simulink model "afe_rst_inv_psm_distributed_control_two_delays"  (R2026a)
settings: Solver=ode1be  StopTime=simlength  FixedStep=tc  MaxStep=Tc
values from neighbouring files (symbols this model uses):
  Amplitude_U = 1.16    [grid_fault_generator.m]
  Amplitude_V = Amplitude_U    (= 1.16)    [grid_fault_generator.m]
  Amplitude_W = Amplitude_U    (= 1.16)    [grid_fault_generator.m]
  end_time_LVRT = start_time_LVRT + error_length    [grid_fault_generator.m]
  Igrid_phase_normalization_factor = 270*sqrt(2)    [grid_emulator.m]
  omega_grid_emulator_nom = w_grid    (= 314.159265359)    [grid_emulator.m]
  omega_grid_nom = w_grid    (= 314.159265359)    [grid_emulator.m]
  t_ramp = 20e-3    (= 0.02)    [grid_fault_generator.m]
  ugrid_factor = 1    [grid_emulator.m]
  V_phase_normalization_factor = Vgrid_phase_normalization_factor    [grid_emulator.m]
  Vdc_bez = 1070    [grid_emulator.m]
  Vemu_ref_norm = Vemu_ref * sqrt(2) / V_phase_normalization_factor    [grid_emulator.m]
  vn_eta_pu = 0    [grid_emulator.m]
  vn_xi_pu = 0    [grid_emulator.m]
  vp_xi_pu = 1    [grid_emulator.m]
undefined symbols (not defined in the file or in its folder): Adrso, Aresd, Bresd, CFi, CFu, Cresd, Crso, CTRPIFF_CLIP_RELEASE, dead_time_INV, emf_fb_p, emf_fb_p_ccaller_1, emf_fb_p_ccaller_2, emf_p, emf_p_ccaller_1, emf_p_ccaller_2, fPWM_INV, g0_161Hz, g0_500Hz, g1_161Hz, g1_500Hz, i_grid_neg_eta_lim, i_grid_neg_eta_red_lim, i_grid_neg_xi_lim, i_grid_neg_xi_red_lim, i_grid_pos_eta_lim, i_grid_pos_eta_red_lim, ibez, id_lim, ieta_neg_ref_lim, ieta_pos_ref_lim, iq_lim, ixi_pos_ref_lim, Jm_norm, k_frt_ref, kg, ki_afe, ki_i, ki_id, ki_iq, ki_rc_neg_grid, ki_rc_pos_grid, ki_vs, ki_w, kp_afe, kp_i, kp_id, kp_iq, kp_rc_neg_grid, kp_rc_pos_grid, kp_vs, kp_w, kw, l1, l2, Lalpha_norm, Ld_norm, Ldrso, Lq_norm, Ls_norm, luenberger_l1 ... (+30)
libraries: fl_lib x146, nesl_utility x62, simulink x8, cstblocks_lti x7, sl_discontinuities x3, single_phase_transformer_lib x3, flexshaft_lib x1, permanent_magnet_synchronous_machine x1
(part 1 of 14)
settings Model: SimulationMode=accelerator  Creator=dbagn  LastModifiedBy=dbagn
settings SolverCC: NumberNewtonIterations=3.0  ZeroCrossControl=DisableAll  SolverResetMethod=Robust
settings SFSimCC: SimUserIncludeDirs=include  CustomCodeUndefinedFunction=ThrowError
settings SFSimCC: SimCustomHeaderCode=|
  | #include "mavgflt.h"
  | #include "mavgflt_simulink.h"
  | #include "bemf_obsv_load_est.h"
  | #include "bemf_obsv.h"
  | #include "bemf_obsv_simulink.h"
  | #include "dqvector_pi.h"
  | #include "dqvector_pi_simulink.h"
  | #include "bemf_obsv_load_est_simulink.h"
  | #include "sv_pwm.h"
  | #include "sv_pwm_simulink.h"
settings SFSimCC: SimUserSources=|
  | "mavgflt_simulink.c"
  | "mavgflt.c"
  | "bemf_obsv_simulink.c"
  | "bemf_obsv.c"
  | "bemf_obsv_load_est_simulink.c"
  | "bemf_obsv_load_est.c"
  | "dqvector_pi.c"
  | "dqvector_pi_simulink.c"
  | "sv_pwm_simulink.c"
  | "sv_pwm.c"
settings SimscapeCC: SimscapeNominalValues="[{\"value\":\"1\",\"unit\":\"A\"},{\"value\":\"1\",\"unit\":\"bar\"},{\"value\":\"1\",\"unit\":\"cm^2\"},{\"value\":\"1\",\"unit\":\"cm^3/s\"},{\"value\":\"1\",\"unit\":\"kJ/kg\"},{\"value\":\"1\",\"unit\":\"kW\"},{\"value\":\"1\",\"unit\":\"l\"},{\"value\":\"1\",\"unit\":\"N\"},{\"value\":\"1\",\"unit\":\"N*m\"},{\"value\":\"1\",\"unit\":\"V\"}]"  SimscapeLogType=none  SimscapeLogDataHistory=5000.0

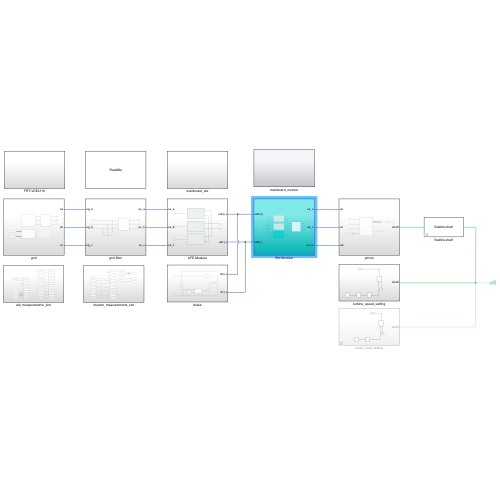
[thumbnail: Simulink's stored preview of the top-level diagram]
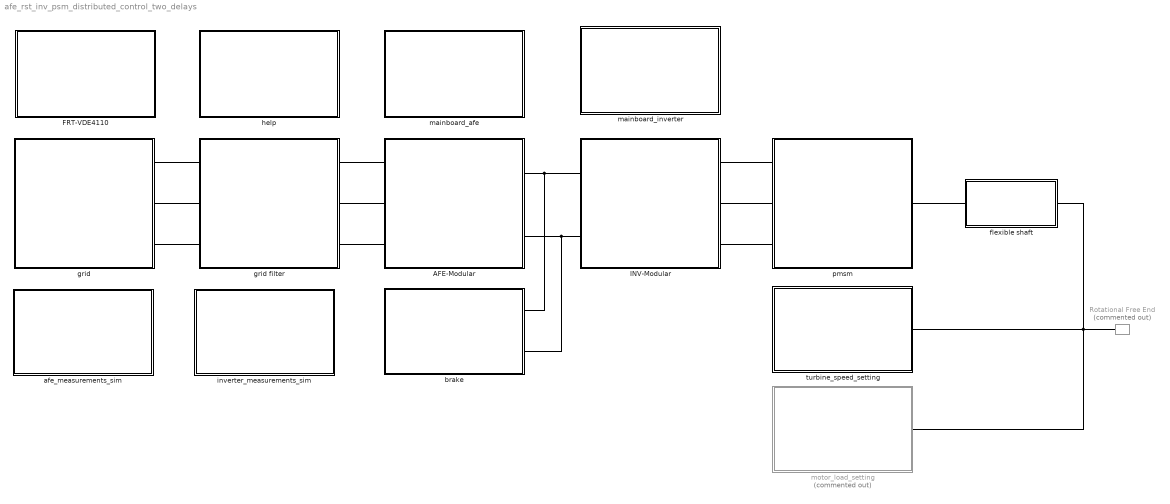
== system afe_rst_inv_psm_distributed_control_two_delays ==
  AFE-Modular : Subsystem
  FRT-VDE4110 : Subsystem
  INV-Modular : Subsystem
  Rotational Free End : fl_lib/Mechanical/Rotational Elements/Rotational Free End  Commented=on  w_specify=off  w_priority=None  w=0 rad/s  w_nominal_specify=off  w_nominal_value=1  w_nominal_unit=rad/s
  afe_measurements_sim : Subsystem
  brake : Subsystem
  flexible shaft : Subsystem
      mask Display: disp('flexible shaft')
  grid : Subsystem
  grid filter : Subsystem
  help : Subsystem
      mask Display: disp('ReadMe')
  inverter_measurements_sim : Subsystem
  mainboard_afe : Subsystem
  mainboard_inverter : Subsystem
  motor_load_setting : Subsystem  Commented=on
  pmsm : Subsystem
  turbine_speed_setting : Subsystem
  connections:
  grid/RConn1 -- grid filter/RConn1
  grid/RConn2 -- grid filter/RConn2
  grid/RConn3 -- grid filter/RConn3
  Rotational Free End/LConn1 -- turbine_speed_setting/LConn1 -- motor_load_setting/LConn1 -- flexible shaft/RConn1
  AFE-Modular/LConn2 -- grid filter/LConn2
  grid filter/LConn1 -- AFE-Modular/LConn1
  grid filter/LConn3 -- AFE-Modular/LConn3
  AFE-Modular/RConn1 -- INV-Modular/RConn1 -- brake/LConn1
  AFE-Modular/RConn2 -- INV-Modular/RConn2 -- brake/LConn2
  INV-Modular/LConn1 -- pmsm/LConn1
  INV-Modular/LConn2 -- pmsm/LConn2
  INV-Modular/LConn3 -- pmsm/LConn3
  pmsm/RConn1 -- flexible shaft/LConn1

== system afe_rst_inv_psm_distributed_control_two_delays/AFE-Modular ==
  afe_leg_a : Subsystem
  afe_leg_b : Subsystem
  afe_leg_c : Subsystem
  us_a : PMIOPort  Side=Left
  us_b : PMIOPort  Port=2  Side=Left
  us_c : PMIOPort  Port=3  Side=Left
  udc(+) : PMIOPort  Port=4  Side=Right
  udc(-) : PMIOPort  Port=5  Side=Right
  connections:
  afe_leg_c/LConn1 -- us_c/RConn1
  afe_leg_a/RConn1 -- udc(+)/RConn1 -- afe_leg_b/RConn1 -- afe_leg_c/RConn1
  afe_leg_a/RConn2 -- udc(-)/RConn1 -- afe_leg_b/RConn2 -- afe_leg_c/RConn2
  afe_leg_b/LConn1 -- us_b/RConn1
  afe_leg_a/LConn1 -- us_a/RConn1

== system afe_rst_inv_psm_distributed_control_two_delays/FRT-VDE4110 ==
  FRT-Detection : Subsystem
  FRT-PosNegReactiveCurrentReferences : Subsystem
  frt_detection : Scope  NumInputPorts=3
      settings: SampleTime=ts_afe  ActiveDisplayYMinimum=-1  ActiveDisplayYMaximum=1
  tag scope: frt_active=global, pwr_lim_enable=global
  wires:
  [v_grid_pos_xi_avg] -> FRT-PosNegReactiveCurrentReferences/1(In1)
  [v_grid_neg_xi_avg] -> FRT-PosNegReactiveCurrentReferences/3(In3)
  [v_grid_neg_eta_avg] -> FRT-PosNegReactiveCurrentReferences/4(In4)
  [v_grid_pos_eta_avg] -> FRT-PosNegReactiveCurrentReferences/2(In2)
  FRT-Detection/3(frt_active) -> [frt_active], frt_detection/2  "frt_active"
  FRT-Detection/4(pwr_lim_enable) -> [pwr_lim_enable], frt_detection/3  "pwr_lim_enable"
  FRT-Detection/2(frt_state) -> frt_detection/1  "frt_state"

== system afe_rst_inv_psm_distributed_control_two_delays/INV-Modular ==
  inv_leg_u : Subsystem
  inv_leg_v : Subsystem
  inv_leg_w : Subsystem
  threephase_vi_measures : Subsystem
  us_u : PMIOPort  Side=Left
  us_v : PMIOPort  Port=2  Side=Left
  us_w : PMIOPort  Port=3  Side=Left
  udc(+) : PMIOPort  Port=4  Side=Right
  udc(-) : PMIOPort  Port=5  Side=Right
  connections:
  inv_leg_w/RConn2 -- udc(-)/RConn1 -- inv_leg_v/RConn2 -- inv_leg_u/RConn2
  inv_leg_w/RConn1 -- inv_leg_u/RConn1 -- udc(+)/RConn1 -- inv_leg_v/RConn1
  threephase_vi_measures/LConn2 -- inv_leg_v/LConn1
  inv_leg_u/LConn1 -- threephase_vi_measures/LConn1
  inv_leg_w/LConn1 -- threephase_vi_measures/LConn3
  us_u/RConn1 -- threephase_vi_measures/RConn1
  us_v/RConn1 -- threephase_vi_measures/RConn2
  threephase_vi_measures/RConn3 -- us_w/RConn1

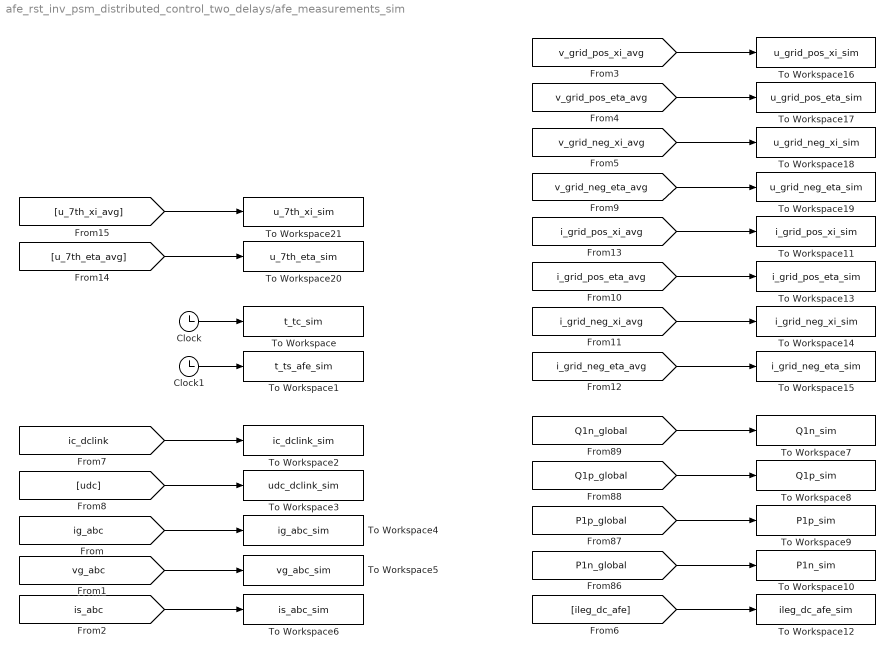
== system afe_rst_inv_psm_distributed_control_two_delays/afe_measurements_sim ==
  Clock : Clock
  Clock1 : Clock
  To Workspace : ToWorkspace  VariableName=t_tc_sim  SampleTime=tc
      settings: MaxDataPoints=Nc
  To Workspace1 : ToWorkspace  VariableName=t_ts_afe_sim  SampleTime=ts_afe
      settings: MaxDataPoints=Ns_afe
  To Workspace10 : ToWorkspace  VariableName=P1n_sim  SampleTime=ts_afe
      settings: MaxDataPoints=Ns_afe
  To Workspace11 : ToWorkspace  VariableName=i_grid_pos_xi_sim  SampleTime=ts_afe
      settings: MaxDataPoints=Ns_afe
  To Workspace12 : ToWorkspace  VariableName=ileg_dc_afe_sim  SampleTime=tc
      settings: MaxDataPoints=Nc
  To Workspace13 : ToWorkspace  VariableName=i_grid_pos_eta_sim  SampleTime=ts_afe
      settings: MaxDataPoints=Ns_afe
  To Workspace14 : ToWorkspace  VariableName=i_grid_neg_xi_sim  SampleTime=ts_afe
      settings: MaxDataPoints=Ns_afe
  To Workspace15 : ToWorkspace  VariableName=i_grid_neg_eta_sim  SampleTime=ts_afe
      settings: MaxDataPoints=Ns_afe
  To Workspace16 : ToWorkspace  VariableName=u_grid_pos_xi_sim  SampleTime=ts_afe
      settings: MaxDataPoints=Ns_afe
  To Workspace17 : ToWorkspace  VariableName=u_grid_pos_eta_sim  SampleTime=ts_afe
      settings: MaxDataPoints=Ns_afe
  To Workspace18 : ToWorkspace  VariableName=u_grid_neg_xi_sim  SampleTime=ts_afe
      settings: MaxDataPoints=Ns_afe
  To Workspace19 : ToWorkspace  VariableName=u_grid_neg_eta_sim  SampleTime=ts_afe
      settings: MaxDataPoints=Ns_afe
  To Workspace2 : ToWorkspace  VariableName=ic_dclink_sim  SampleTime=tc
      settings: MaxDataPoints=Nc
  To Workspace20 : ToWorkspace  VariableName=u_7th_eta_sim  SampleTime=ts_afe
      settings: MaxDataPoints=Ns_afe
  To Workspace21 : ToWorkspace  VariableName=u_7th_xi_sim  SampleTime=ts_afe
      settings: MaxDataPoints=Ns_afe
  To Workspace3 : ToWorkspace  VariableName=udc_dclink_sim  SampleTime=tc
      settings: MaxDataPoints=Nc
  To Workspace4 : ToWorkspace  VariableName=ig_abc_sim  SampleTime=tc
      settings: MaxDataPoints=Nc
  To Workspace5 : ToWorkspace  VariableName=vg_abc_sim  SampleTime=tc
      settings: MaxDataPoints=Nc
  To Workspace6 : ToWorkspace  VariableName=is_abc_sim  SampleTime=tc
      settings: MaxDataPoints=Nc
  To Workspace7 : ToWorkspace  VariableName=Q1n_sim  SampleTime=ts_afe
      settings: MaxDataPoints=Ns_afe
  To Workspace8 : ToWorkspace  VariableName=Q1p_sim  SampleTime=ts_afe
      settings: MaxDataPoints=Ns_afe
  To Workspace9 : ToWorkspace  VariableName=P1p_sim  SampleTime=ts_afe
      settings: MaxDataPoints=Ns_afe
  wires:
  Clock1/1 -> To Workspace1/1
  Clock/1 -> To Workspace/1
  [ic_dclink] -> To Workspace2/1
  [udc] -> To Workspace3/1
  [ig_abc] -> To Workspace4/1
  [vg_abc] -> To Workspace5/1
  [is_abc] -> To Workspace6/1
  [Q1n_global] -> To Workspace7/1
  [Q1p_global] -> To Workspace8/1
  [P1p_global] -> To Workspace9/1
  [P1n_global] -> To Workspace10/1
  [ileg_dc_afe] -> To Workspace12/1
  [i_grid_pos_xi_avg] -> To Workspace11/1
  [i_grid_pos_eta_avg] -> To Workspace13/1
  [i_grid_neg_xi_avg] -> To Workspace14/1
  [i_grid_neg_eta_avg] -> To Workspace15/1
  [v_grid_pos_xi_avg] -> To Workspace16/1
  [v_grid_pos_eta_avg] -> To Workspace17/1
  [v_grid_neg_xi_avg] -> To Workspace18/1
  [v_grid_neg_eta_avg] -> To Workspace19/1
  [u_7th_eta_avg] -> To Workspace20/1
  [u_7th_xi_avg] -> To Workspace21/1

== system afe_rst_inv_psm_distributed_control_two_delays/brake ==
  Constant1 : Constant  Value=Vdc_ref
  MATLAB Function : MATLAB Function  TreatAsAtomicUnit=on
  PS-Simulink Converter : nesl_utility/PS-Simulink Converter  PhysicalDomain=network_engine_domain  SubClassName=ps_output  LeftPortType=input  RightPortType=output  PseudoPeriodic=off  Frequencies=[]  VectorFormat=1-D array  Unit=V  AffineConversion=off
  Resistor : fl_lib/Electrical/Electrical Elements/Resistor  R=2.5 Ohm  i_specify=off  i_priority=None  i=0 A  i_nominal_specify=off  i_nominal_value=1  i_nominal_unit=A  v_specify=off  v_priority=None  v=0 V  v_nominal_specify=off  v_nominal_value=1  v_nominal_unit=V
  Simulink-PS Converter4 : nesl_utility/Simulink-PS Converter  PhysicalDomain=network_engine_domain  SubClassName=ps_input  LeftPortType=input  RightPortType=output  PseudoPeriodic=off  Frequencies=[]  NoiseDistribution=none  NoiseParameters=[]  Unit=1  AffineConversion=on  FilteringAndDerivatives=provide  SimscapeFilterOrder=1  InputFilterTimeConstant=0.001  UdotUserProvided=0
  Unit Delay : UnitDelay  SampleTime=ts_afe
  Voltage Sensor : fl_lib/Electrical/Electrical Sensors/Voltage Sensor
  switch_5 : Subsystem
      settings: PortSchema="{\"entries\":[{\"content\":{\"sides\":[{\"content\":{\"connectorIds\":[\"LConn1\"]},\"type\":\"ConnectorPlacement.EquallySpacedRectSide\",\"uuid\":\"9277da8d-d460-43e6-8478-dd662f15d226\"},{\"content\":{\"connectorIds\":[],\"side\":\"RIGHT\"},\"type\":\"ConnectorPlacement.EquallySpacedRectSide\",\"uuid\":\"a7ece396-f1d9-4f4f-a05b-db1fc65d6e1d\"},{\"content\":{\"connectorIds\":[\"LConn2\"],\"side\":\"TOP\"},\"type\":\"ConnectorPlacement.EquallySpacedRectSide\",\"uuid\":\"fdd70777-e9cf-4317-afb6-cae87f75d5b0\"},{\"content\":{\"connectorIds\":[\"RConn1\"],\"side\":\"BOTTOM\"},\"type\":\"ConnectorPlacement.EquallySpacedRectSide\",\"uuid\":\"2353ed68-b1a1-4775-9ca9-31e268d5443b\"}]},\"type\":\"ConnectorPlacement.EquallySpacedConnector\",\"uuid\":\"d5479f4c-4e65-4791-adcb-73df11f88590\"}],\"packageUris\":[\"http://schema.mathworks.com/mf0/Connector/R2020b\"],\"version\":\"1.0\"}"
  switch_6 : Subsystem
      settings: PortSchema="{\"entries\":[{\"content\":{\"sides\":[{\"content\":{},\"type\":\"ConnectorPlacement.EquallySpacedRectSide\",\"uuid\":\"9277da8d-d460-43e6-8478-dd662f15d226\"},{\"content\":{\"side\":\"RIGHT\"},\"type\":\"ConnectorPlacement.EquallySpacedRectSide\",\"uuid\":\"a7ece396-f1d9-4f4f-a05b-db1fc65d6e1d\"},{\"content\":{\"connectorIds\":[\"LConn1\"],\"side\":\"TOP\"},\"type\":\"ConnectorPlacement.EquallySpacedRectSide\",\"uuid\":\"fdd70777-e9cf-4317-afb6-cae87f75d5b0\"},{\"content\":{\"connectorIds\":[\"RConn1\"],\"side\":\"BOTTOM\"},\"type\":\"ConnectorPlacement.EquallySpacedRectSide\",\"uuid\":\"2353ed68-b1a1-4775-9ca9-31e268d5443b\"}]},\"type\":\"ConnectorPlacement.EquallySpacedConnector\",\"uuid\":\"d5479f4c-4e65-4791-adcb-73df11f88590\"}],\"packageUris\":[\"http://schema.mathworks.com/mf0/Connector/R2020b\"],\"version\":\"1.0\"}"
  dc(+) : PMIOPort  Side=Left
  dc(-) : PMIOPort  Port=2  Side=Left
  wires:
  Unit Delay/1 -> Simulink-PS Converter4/1
  Constant1/1 -> MATLAB Function/2(udc_ref)
  PS-Simulink Converter/1 -> MATLAB Function/1(u)
  MATLAB Function/1(y) -> Unit Delay/1
  connections:
  dc(-)/RConn1 -- switch_5/RConn1 -- Voltage Sensor/RConn2
  Voltage Sensor/LConn1 -- switch_6/LConn1 -- Resistor/LConn1 -- dc(+)/RConn1
  PS-Simulink Converter/LConn1 -- Voltage Sensor/RConn1
  switch_5/LConn1 -- Simulink-PS Converter4/RConn1
  switch_6/RConn1 -- switch_5/LConn2 -- Resistor/RConn1

== system afe_rst_inv_psm_distributed_control_two_delays/flexible shaft ==
  flexible shaft : flexshaft_lib/flexible shaft  b1=0 N*m*s/rad  J1=1e-4 kg*m^2  b2=0 N*m*s/rad  J2=1e-4 kg*m^2  b_theta=0 N*m*s/rad  k_theta=1e12 N*m/rad  w_1_specify=off  w_1_priority=None  w_1=0 rad/s  w_1_nominal_specify=off  w_1_nominal_value=1  w_1_nominal_unit=rad/s  w_2_specify=off  w_2_priority=None  w_2=0 rad/s  w_2_nominal_specify=off  w_2_nominal_value=1  w_2_nominal_unit=rad/s  t_1_specify=off  t_1_priority=None  t_1=0 N*m  t_1_nominal_specify=off  t_1_nominal_value=1  t_1_nominal_unit=N*m  t_2_specify=off  t_2_priority=None  t_2=0 N*m  t_2_nominal_specify=off  t_2_nominal_value=1  t_2_nominal_unit=N*m  t_theta_specify=off  t_theta_priority=None  t_theta=0 N*m  t_theta_nominal_specify=off  t_theta_nominal_value=1  t_theta_nominal_unit=N*m
  s2 : PMIOPort  Side=Right
  s1 : PMIOPort  Port=2  Side=Left
  connections:
  flexible shaft/RConn1 -- s2/RConn1
  flexible shaft/LConn1 -- s1/RConn1

== system afe_rst_inv_psm_distributed_control_two_delays/grid ==
  grid_emulator : Subsystem
  instantaneus_power : Subsystem
  sequences accordind to VDE411 : Subsystem  Commented=on
  threephase_vi_measures : Subsystem
  ua : PMIOPort  Side=Right
  ub : PMIOPort  Port=2  Side=Right
  uc : PMIOPort  Port=3  Side=Right
  wires:
  [vg_abc] -> instantaneus_power/1(Vline)
  [ig_abc] -> instantaneus_power/2(Iline)
  connections:
  threephase_vi_measures/LConn3 -- grid_emulator/RConn3
  threephase_vi_measures/LConn1 -- grid_emulator/RConn1
  threephase_vi_measures/RConn2 -- ub/RConn1
  threephase_vi_measures/LConn2 -- grid_emulator/RConn2
  threephase_vi_measures/RConn1 -- ua/RConn1
  threephase_vi_measures/RConn3 -- uc/RConn1

== system afe_rst_inv_psm_distributed_control_two_delays/grid filter ==
  CFu1 : fl_lib/Electrical/Electrical Elements/Capacitor  c=CFu F  r=RCFu Ohm  g=0 1/Ohm  i_specify=off  i_priority=None  i=0 A  i_nominal_specify=off  i_nominal_value=1  i_nominal_unit=A  v_specify=off  v_priority=None  v=0 V  v_nominal_specify=off  v_nominal_value=1  v_nominal_unit=V  vc_specify=off  vc_priority=High  vc=0 V  vc_nominal_specify=off  vc_nominal_value=1  vc_nominal_unit=V
  CFu2 : fl_lib/Electrical/Electrical Elements/Capacitor  c=CFu F  r=RCFu Ohm  g=0 1/Ohm  i_specify=off  i_priority=None  i=0 A  i_nominal_specify=off  i_nominal_value=1  i_nominal_unit=A  v_specify=off  v_priority=None  v=0 V  v_nominal_specify=off  v_nominal_value=1  v_nominal_unit=V  vc_specify=off  vc_priority=High  vc=0 V  vc_nominal_specify=off  vc_nominal_value=1  vc_nominal_unit=V
  CFu3 : fl_lib/Electrical/Electrical Elements/Capacitor  c=CFu F  r=RCFu Ohm  g=0 1/Ohm  i_specify=off  i_priority=None  i=0 A  i_nominal_specify=off  i_nominal_value=1  i_nominal_unit=A  v_specify=off  v_priority=None  v=0 V  v_nominal_specify=off  v_nominal_value=1  v_nominal_unit=V  vc_specify=off  vc_priority=High  vc=0 V  vc_nominal_specify=off  vc_nominal_value=1  vc_nominal_unit=V
  threephase_vi_measures_stack : Subsystem
  us_a : PMIOPort  Side=Left
  ug_a : PMIOPort  Port=2  Side=Right
  us_b : PMIOPort  Port=3  Side=Left
  ug_b : PMIOPort  Port=4  Side=Right
  us_c : PMIOPort  Port=5  Side=Left
  ug_c : PMIOPort  Port=6  Side=Right
  connections:
  CFu3/RConn1 -- CFu1/RConn1 -- CFu2/RConn1
  CFu1/LConn1 -- threephase_vi_measures_stack/RConn1 -- ug_a/RConn1
  ug_c/RConn1 -- threephase_vi_measures_stack/RConn3 -- CFu3/LConn1
  CFu2/LConn1 -- threephase_vi_measures_stack/RConn2 -- ug_b/RConn1
  threephase_vi_measures_stack/LConn1 -- us_a/RConn1
  threephase_vi_measures_stack/LConn2 -- us_b/RConn1
  threephase_vi_measures_stack/LConn3 -- us_c/RConn1

== system afe_rst_inv_psm_distributed_control_two_delays/help ==

== system afe_rst_inv_psm_distributed_control_two_delays/inverter_measurements_sim ==
  Bus Creator : BusCreator  Inputs=3
  Clock : Clock  Commented=on
  Clock1 : Clock
  Gain : Gain  Gain=psi_bez
  Gain1 : Gain  Gain=psi_bez
  To Workspace : ToWorkspace  Commented=on  VariableName=t_tc_sim  SampleTime=tc
      settings: MaxDataPoints=Nc
  To Workspace1 : ToWorkspace  VariableName=t_ts_inv_sim  SampleTime=ts_inv
      settings: MaxDataPoints=Ns_inv
  To Workspace10 : ToWorkspace  VariableName=rpm_motor_sim  SampleTime=ts_inv
      settings: MaxDataPoints=Ns_inv
  To Workspace11 : ToWorkspace  VariableName=iuvw_sim  SampleTime=tc
      settings: MaxDataPoints=Nc
  To Workspace12 : ToWorkspace  VariableName=ileg_dc_inv_sim  SampleTime=tc
      settings: MaxDataPoints=Nc
  To Workspace13 : ToWorkspace  VariableName=theta_elec_pmsm_sim  SampleTime=ts_inv
      settings: MaxDataPoints=Ns_inv
  To Workspace2 : ToWorkspace  VariableName=ualpha_pu_sim  SampleTime=ts_inv
      settings: MaxDataPoints=Ns_inv
  To Workspace3 : ToWorkspace  VariableName=ubeta_pu_sim  SampleTime=ts_inv
      settings: MaxDataPoints=Ns_inv
  To Workspace4 : ToWorkspace  VariableName=psi_pu_alpha_hat_sim  SampleTime=ts_inv
      settings: MaxDataPoints=Ns_inv
  To Workspace5 : ToWorkspace  VariableName=psi_pu_beta_hat_sim  SampleTime=ts_inv
      settings: MaxDataPoints=Ns_inv
  To Workspace6 : ToWorkspace  VariableName=psi_alpha_hat_sim  SampleTime=ts_inv
      settings: MaxDataPoints=Ns_inv
  To Workspace7 : ToWorkspace  VariableName=psi_alpha_pmsm_sim  SampleTime=ts_inv
      settings: MaxDataPoints=Ns_inv
  To Workspace8 : ToWorkspace  VariableName=psi_beta_hat_sim  SampleTime=ts_inv
      settings: MaxDataPoints=Ns_inv
  To Workspace9 : ToWorkspace  VariableName=psi_beta_pmsm_sim  SampleTime=ts_inv
      settings: MaxDataPoints=Ns_inv
  wires:
  [phi_pu_beta_hat] -> Gain1/1
  Gain1/1 -> To Workspace8/1  "psi_beta_hat"
  [phi_pu_beta_hat] -> To Workspace5/1  "phi_beta_hat"
  [phi_pu_alpha_hat] -> To Workspace4/1  "phi_alpha_hat"
  [ualpha_pu] -> To Workspace2/1
  [phi_alpha_pmsm] -> To Workspace7/1  "phi_alpha"
  Clock1/1 -> To Workspace1/1
  Gain/1 -> To Workspace6/1  "psi_alpha_hat"
  Clock/1 -> To Workspace/1
  [ubeta_pu] -> To Workspace3/1  "ub"
  [phi_pu_alpha_hat] -> Gain/1
  [phi_beta_pmsm] -> To Workspace9/1  "phi_beta"
  [rpm_motor] -> To Workspace10/1
  [iv_pmsm] -> Bus Creator/2  "iv"
  [iw_pmsm] -> Bus Creator/3  "iw"
  [iu_pmsm] -> Bus Creator/1  "iu"
  Bus Creator/1 -> To Workspace11/1
  [theta_elec_pmsm] -> To Workspace13/1  "theta_elec_pmsm"
  [ileg_dc_inv] -> To Workspace12/1

== system afe_rst_inv_psm_distributed_control_two_delays/mainboard_afe ==
  current_sequence_avg : Subsystem
  dq_pll : Subsystem
  grid_current_sampling_and_alpha_beta_transformation : Subsystem
  grid_voltage_sampling_and_alpha_beta_transformation : Subsystem
  ig_alphabeta2xieta : Subsystem
  sequences_current_control : Subsystem
  ug_alphabeta2xieta : Subsystem
  voltage-current-acquisition : Subsystem
  voltage_sequence_avg : Subsystem
  tag scope: i_grid_neg_eta_avg=global, i_grid_neg_xi_avg=global, i_grid_pos_eta_avg=global, i_grid_pos_xi_avg=global, v_grid_neg_eta_avg=global, v_grid_neg_xi_avg=global, v_grid_pos_eta_avg=global, v_grid_pos_xi_avg=global
  wires:
  [gamma_grid_pll] -> ug_alphabeta2xieta/3(gamma), ig_alphabeta2xieta/3(gamma)
  ug_alphabeta2xieta/1(xi) -> voltage_sequence_avg/1(v_grid_pos_xi)  "pos_xi"
  ug_alphabeta2xieta/2(eta) -> voltage_sequence_avg/2(v_grid_pos_eta)  "pos_eta"
  ug_alphabeta2xieta/3(v_grid_neg_xi) -> voltage_sequence_avg/3(v_grid_neg_xi)  "neg_xi"
  ug_alphabeta2xieta/4(v_grid_neg_eta) -> voltage_sequence_avg/4(v_grid_neg_eta)  "neg_eta"
  ig_alphabeta2xieta/1(xi) -> current_sequence_avg/1(i_grid_pos_xi)
  ig_alphabeta2xieta/2(v_grid_pos_eta) -> current_sequence_avg/2(i_grid_pos_eta)
  ig_alphabeta2xieta/3(v_grid_neg_xi) -> current_sequence_avg/3(i_grid_neg_xi)
  ig_alphabeta2xieta/4(e) -> current_sequence_avg/4(i_grid_neg_eta)
  current_sequence_avg/1(i_grid_pos_xi_avg) -> [i_grid_pos_xi_avg], sequences_current_control/1(i_pos_xi)
  current_sequence_avg/2(i_grid_pos_eta_avg) -> [i_grid_pos_eta_avg], sequences_current_control/2(i_pos_eta)
  current_sequence_avg/3(i_grid_neg_xi_avg) -> sequences_current_control/3(i_neg_xi), [i_grid_neg_xi_avg]
  current_sequence_avg/4(i_grid_neg_eta_avg) -> sequences_current_control/4(i_neg_eta), [i_grid_neg_eta_avg]
  grid_voltage_sampling_and_alpha_beta_transformation/1(u_grid_alpha) -> ug_alphabeta2xieta/1(alpha)
  grid_voltage_sampling_and_alpha_beta_transformation/2(u_grid_beta) -> ug_alphabeta2xieta/2(beta)
  grid_current_sampling_and_alpha_beta_transformation/1(i_grid_alpha) -> ig_alphabeta2xieta/1(alpha)
  grid_current_sampling_and_alpha_beta_transformation/2(i_grid_beta) -> ig_alphabeta2xieta/2(beta)
  voltage_sequence_avg/3(v_grid_neg_xi_avg) -> [v_grid_neg_xi_avg]
  voltage_sequence_avg/2(v_grid_pos_eta_avg) -> [v_grid_pos_eta_avg]
  voltage_sequence_avg/1(v_grid_pos_xi_avg) -> [v_grid_pos_xi_avg]
  voltage_sequence_avg/4(v_grid_neg_eta_avg) -> [v_grid_neg_eta_avg]

== system afe_rst_inv_psm_distributed_control_two_delays/mainboard_inverter ==
  Gain : Gain  Gain=1/omega_bez
  Unit Delay : UnitDelay  SampleTime=ts_inv
  Zero-Order Hold : ZeroOrderHold  SampleTime=ts_inv
  double_integrator_observer : Subsystem
  motor_phases : Scope  NumInputPorts=4
      settings: SampleTime=tc  ActiveDisplayYMinimum=-3.92699  ActiveDisplayYMaximum=3.92698
  motor_phases_encoder : Scope  NumInputPorts=4
      settings: SampleTime=tc  ActiveDisplayYMinimum=-3.92699  ActiveDisplayYMaximum=3.92699
  motor_speed_hat : Scope  NumInputPorts=4
      settings: SampleTime=tc  ActiveDisplayYMinimum=-0.12512  ActiveDisplayYMaximum=1.1261  DataLoggingVariableName=ScopeData3
  tag scope: motor_phase_mb=global, motor_speed_pu_mb=global
  wires:
  [motor_theta_hat_dbu] -> motor_phases/1  "motor_phase_hat_dbu"
  [motor_theta_hat_dbv] -> motor_phases/2  "motor_phase_hat_dbv"
  [motor_theta_hat_dbw] -> motor_phases/3  "motor_phase_hat_dbw"
  [theta_elec_pmsm] -> motor_phases/4  "motor_phase_psm"
  [theta_elec_pmsm] -> motor_phases_encoder/4  "motor_phase_psm"
  [motor_phase_mb_fb_dbw_luenberger] -> motor_phases_encoder/3  "motor_phase_hat_dbw"
  [motor_phase_mb_fb_dbv_luenberger] -> motor_phases_encoder/2  "motor_phase_hat_dbv"
  [motor_phase_mb_fb_dbu_luenberger] -> motor_phases_encoder/1  "motor_phase_hat_dbu"
  Zero-Order Hold/1 -> Unit Delay/1
  [theta_elec_pmsm] -> Zero-Order Hold/1
  Unit Delay/1 -> double_integrator_observer/1(theta)
  double_integrator_observer/1(omega_pu_hat) -> [motor_speed_pu_mb]
  double_integrator_observer/2(theta_hat) -> [motor_phase_mb]  "theta_hat"
  [omega_elec_pmsm] -> Gain/1
  [motor_omega_hat_pu_dbw] -> motor_speed_hat/3  "motor_omega_hat_dbw"
  [motor_omega_hat_pu_dbv] -> motor_speed_hat/2  "motor_omega_hat_dbv"
  [motor_omega_hat_pu_dbu] -> motor_speed_hat/1  "motor_omega_hat_dbu"
  Gain/1 -> motor_speed_hat/4  "motor_omega_psm"

== system afe_rst_inv_psm_distributed_control_two_delays/motor_load_setting ==
  Ideal Torque Source : fl_lib/Mechanical/Mechanical Sources/Ideal Torque Source
  Mechanical Rotational Reference : fl_lib/Mechanical/Rotational Elements/Mechanical Rotational Reference
  PS Step : fl_lib/Physical Signals/Sources/PS Step  step_time=0.5 s  initial_value=1 N*m  final_value=1 N*m
  PS Transfer Function : fl_lib/Physical Signals/Linear Operators/PS Transfer Function  transfer_function_type=foundation.enum.transfer_function_type.lag  T=1 s  T1=2 s  T2=1 s  reset_method=foundation.enum.IntegratorResetSpec.None  initial_condition_spec=foundation.enum.IntegratorICSpec.Internal  y0=0 N*m
  shaft : PMIOPort  Side=Left
  connections:
  Ideal Torque Source/LConn1 -- shaft/RConn1
  Ideal Torque Source/RConn2 -- Mechanical Rotational Reference/LConn1
  PS Transfer Function/RConn1 -- Ideal Torque Source/RConn1
  PS Step/RConn1 -- PS Transfer Function/LConn1

== system afe_rst_inv_psm_distributed_control_two_delays/pmsm ==
  Bus Selector : BusSelector  OutputSignals=omega_mech (rpm)
  Constant : Constant  Value=psi_m
  Simulink-PS Converter3 : nesl_utility/Simulink-PS Converter  PhysicalDomain=network_engine_domain  SubClassName=ps_input  LeftPortType=input  RightPortType=output  PseudoPeriodic=off  Frequencies=[]  NoiseDistribution=none  NoiseParameters=[]  Unit=V*s  AffineConversion=on  FilteringAndDerivatives=provide  SimscapeFilterOrder=1  InputFilterTimeConstant=0.001  UdotUserProvided=0
  synchronous_motor : Subsystem
  uu : PMIOPort  Side=Left
  uv : PMIOPort  Port=2  Side=Left
  uw : PMIOPort  Port=3  Side=Left
  shaft : PMIOPort  Port=4  Side=Right
  tag scope: rpm_motor=global
  wires:
  synchronous_motor/1(motor_data) -> Bus Selector/1
  Bus Selector/1 -> [rpm_motor]  "<omega_mech (rpm)>"
  Constant/1 -> Simulink-PS Converter3/1
  connections:
  synchronous_motor/LConn1 -- uu/RConn1
  synchronous_motor/LConn4 -- Simulink-PS Converter3/RConn1
  synchronous_motor/LConn3 -- uw/RConn1
  synchronous_motor/LConn2 -- uv/RConn1
  synchronous_motor/RConn1 -- shaft/RConn1

== system afe_rst_inv_psm_distributed_control_two_delays/turbine_speed_setting ==
  Ideal Angular Velocity Source : fl_lib/Mechanical/Mechanical Sources/Ideal Angular Velocity Source
  Mechanical Rotational Reference : fl_lib/Mechanical/Rotational Elements/Mechanical Rotational Reference
  PS Ramp : fl_lib/Physical Signals/Sources/PS Ramp  slope=omega_m_bez rad/s^2  start_time=0 s  initial_output=0 rad/s  ZeroCross=true
  PS Saturation : fl_lib/Physical Signals/Nonlinear Operators/PS Saturation  upper_limit=omega_m_bez rad/s  lower_limit=-omega_m_bez rad/s  ZeroCross=true
  PS Transfer Function : fl_lib/Physical Signals/Linear Operators/PS Transfer Function  transfer_function_type=foundation.enum.transfer_function_type.lag  T=0.1 s  T1=2 s  T2=1 s  reset_method=foundation.enum.IntegratorResetSpec.None  initial_condition_spec=foundation.enum.IntegratorICSpec.Internal  y0=0 rad/s
  shaft : PMIOPort  Side=Left
  connections:
  Mechanical Rotational Reference/LConn1 -- Ideal Angular Velocity Source/RConn2
  Ideal Angular Velocity Source/LConn1 -- shaft/RConn1
  PS Transfer Function/RConn1 -- Ideal Angular Velocity Source/RConn1
  PS Saturation/LConn1 -- PS Ramp/RConn1
  PS Saturation/RConn1 -- PS Transfer Function/LConn1

== system afe_rst_inv_psm_distributed_control_two_delays/AFE-Modular/afe_leg_a ==
  Capacitor : fl_lib/Electrical/Electrical Elements/Capacitor  c=CFi/3 F  r=0.2e-3 Ohm  g=0 1/Ohm  i_specify=off  i_priority=None  i=0 A  i_nominal_specify=off  i_nominal_value=1  i_nominal_unit=A  v_specify=on  v_priority=High  v=Vdc_bez V  v_nominal_specify=off  v_nominal_value=1  v_nominal_unit=V  vc_specify=on  vc_priority=High  vc=Vdc_bez V  vc_nominal_specify=off  vc_nominal_value=1  vc_nominal_unit=V
  Current Sensor : fl_lib/Electrical/Electrical Sensors/Current Sensor
  Current Sensor1 : fl_lib/Electrical/Electrical Sensors/Current Sensor
  Electrical Reference : fl_lib/Electrical/Electrical Elements/Electrical Reference
  LFu1 : fl_lib/Electrical/Electrical Elements/Inductor  l=LFu1_AFE H  r=RLFu1_AFE Ohm  g=1e-9 1/Ohm  i_specify=on  i_priority=High  i=0 A  i_nominal_specify=off  i_nominal_value=1  i_nominal_unit=A  v_specify=off  v_priority=None  v=0 V  v_nominal_specify=off  v_nominal_value=1  v_nominal_unit=V  i_L_specify=off  i_L_priority=High  i_L=0 A  i_L_nominal_specify=off  i_L_nominal_value=1  i_L_nominal_unit=A
  Voltage Sensor1 : fl_lib/Electrical/Electrical Sensors/Voltage Sensor
  Voltage Sensor2 : fl_lib/Electrical/Electrical Sensors/Voltage Sensor
  dclink_measure : Subsystem
  driver_board_a : Subsystem
  ic_dclink : nesl_utility/PS-Simulink Converter  PhysicalDomain=network_engine_domain  SubClassName=ps_output  LeftPortType=input  RightPortType=output  PseudoPeriodic=off  Frequencies=[]  VectorFormat=1-D array  Unit=A  AffineConversion=on
  isa_afe : nesl_utility/PS-Simulink Converter  PhysicalDomain=network_engine_domain  SubClassName=ps_output  LeftPortType=input  RightPortType=output  PseudoPeriodic=off  Frequencies=[]  VectorFormat=1-D array  Unit=A  AffineConversion=off
  modulator : Subsystem
  solid_state_inverter : Subsystem
  ug_phase_a_afe : nesl_utility/PS-Simulink Converter  PhysicalDomain=network_engine_domain  SubClassName=ps_output  LeftPortType=input  RightPortType=output  PseudoPeriodic=off  Frequencies=[]  VectorFormat=1-D array  Unit=V  AffineConversion=off
  ug_a : PMIOPort  Side=Left
  Udc(+) : PMIOPort  Port=2  Side=Right
  Udc(-) : PMIOPort  Port=3  Side=Right
  tag scope: ic_dclink=global, isa_dba=global, uga_dba=global
  wires:
  ic_dclink/1 -> [ic_dclink]
  driver_board_a/1(us_alphabeta_ctrl) -> modulator/1(us_alphabeta_ctrl)
  isa_afe/1 -> [isa_dba]  "isa_afe"
  ug_phase_a_afe/1 -> [uga_dba]  "ug_phase_a_afe"
  connections:
  Voltage Sensor2/RConn1 -- dclink_measure/LConn1
  Current Sensor/RConn2 -- Capacitor/LConn1
  Current Sensor/RConn1 -- ic_dclink/LConn1
  Voltage Sensor2/LConn1 -- Current Sensor/LConn1 -- Udc(+)/RConn1 -- solid_state_inverter/LConn1
  Capacitor/RConn1 -- Udc(-)/RConn1 -- solid_state_inverter/LConn2 -- Voltage Sensor2/RConn2
  LFu1/LConn1 -- Voltage Sensor1/LConn1 -- ug_a/RConn1
  Current Sensor1/LConn1 -- solid_state_inverter/RConn1
  Current Sensor1/RConn2 -- LFu1/RConn1
  isa_afe/LConn1 -- Current Sensor1/RConn1
  Electrical Reference/LConn1 -- Voltage Sensor1/RConn2
  Voltage Sensor1/RConn1 -- ug_phase_a_afe/LConn1

== system afe_rst_inv_psm_distributed_control_two_delays/AFE-Modular/afe_leg_b ==
  Capacitor : fl_lib/Electrical/Electrical Elements/Capacitor  c=CFi/3 F  r=0.2e-3 Ohm  g=0 1/Ohm  i_specify=off  i_priority=None  i=0 A  i_nominal_specify=off  i_nominal_value=1  i_nominal_unit=A  v_specify=on  v_priority=High  v=Vdc_bez V  v_nominal_specify=off  v_nominal_value=1  v_nominal_unit=V  vc_specify=on  vc_priority=High  vc=Vdc_bez V  vc_nominal_specify=off  vc_nominal_value=1  vc_nominal_unit=V
  Current Sensor1 : fl_lib/Electrical/Electrical Sensors/Current Sensor
  Electrical Reference : fl_lib/Electrical/Electrical Elements/Electrical Reference
  LFu2 : fl_lib/Electrical/Electrical Elements/Inductor  l=LFu1_AFE H  r=RLFu1_AFE Ohm  g=1e-9 1/Ohm  i_specify=on  i_priority=High  i=0 A  i_nominal_specify=off  i_nominal_value=1  i_nominal_unit=A  v_specify=off  v_priority=None  v=0 V  v_nominal_specify=off  v_nominal_value=1  v_nominal_unit=V  i_L_specify=off  i_L_priority=High  i_L=0 A  i_L_nominal_specify=off  i_L_nominal_value=1  i_L_nominal_unit=A
  Voltage Sensor1 : fl_lib/Electrical/Electrical Sensors/Voltage Sensor
  Voltage Sensor2 : fl_lib/Electrical/Electrical Sensors/Voltage Sensor
  dclink_measure : Subsystem
  driver_board_b : Subsystem
  isb_dbb : nesl_utility/PS-Simulink Converter  PhysicalDomain=network_engine_domain  SubClassName=ps_output  LeftPortType=input  RightPortType=output  PseudoPeriodic=off  Frequencies=[]  VectorFormat=1-D array  Unit=A  AffineConversion=off
  modulator : Subsystem
  solid_state_inverter : Subsystem
  ugb_dbb : nesl_utility/PS-Simulink Converter  PhysicalDomain=network_engine_domain  SubClassName=ps_output  LeftPortType=input  RightPortType=output  PseudoPeriodic=off  Frequencies=[]  VectorFormat=1-D array  Unit=V  AffineConversion=off
  us_b : PMIOPort  Side=Left
  Udc(+) : PMIOPort  Port=2  Side=Right
  Udc(-) : PMIOPort  Port=3  Side=Right
  tag scope: isb_dbb=global, ugb_dbb=global
  wires:
  driver_board_b/1(us_alphabeta_ctrl) -> modulator/1(us_alphabeta_ctrl)
  ugb_dbb/1 -> [ugb_dbb]  "ugb_dbb"
  isb_dbb/1 -> [isb_dbb]  "isb_dbb"
  connections:
  solid_state_inverter/LConn2 -- Udc(-)/RConn1 -- Capacitor/RConn1 -- Voltage Sensor2/RConn2
  solid_state_inverter/LConn1 -- Capacitor/LConn1 -- Udc(+)/RConn1 -- Voltage Sensor2/LConn1
  Voltage Sensor2/RConn1 -- dclink_measure/LConn1
  LFu2/LConn1 -- us_b/RConn1 -- Voltage Sensor1/LConn1
  isb_dbb/LConn1 -- Current Sensor1/RConn1
  Electrical Reference/LConn1 -- Voltage Sensor1/RConn2
  Current Sensor1/LConn1 -- solid_state_inverter/RConn1
  Voltage Sensor1/RConn1 -- ugb_dbb/LConn1
  LFu2/RConn1 -- Current Sensor1/RConn2

== system afe_rst_inv_psm_distributed_control_two_delays/AFE-Modular/afe_leg_c ==
  Capacitor : fl_lib/Electrical/Electrical Elements/Capacitor  c=CFi/3 F  r=0.2e-3 Ohm  g=0 1/Ohm  i_specify=off  i_priority=None  i=0 A  i_nominal_specify=off  i_nominal_value=1  i_nominal_unit=A  v_specify=on  v_priority=High  v=Vdc_bez V  v_nominal_specify=off  v_nominal_value=1  v_nominal_unit=V  vc_specify=on  vc_priority=High  vc=Vdc_bez V  vc_nominal_specify=off  vc_nominal_value=1  vc_nominal_unit=V
  Current Sensor1 : fl_lib/Electrical/Electrical Sensors/Current Sensor
  Electrical Reference : fl_lib/Electrical/Electrical Elements/Electrical Reference
  LFu3 : fl_lib/Electrical/Electrical Elements/Inductor  l=LFu1_AFE H  r=RLFu1_AFE Ohm  g=1e-9 1/Ohm  i_specify=on  i_priority=High  i=0 A  i_nominal_specify=off  i_nominal_value=1  i_nominal_unit=A  v_specify=off  v_priority=None  v=0 V  v_nominal_specify=off  v_nominal_value=1  v_nominal_unit=V  i_L_specify=off  i_L_priority=High  i_L=0 A  i_L_nominal_specify=off  i_L_nominal_value=1  i_L_nominal_unit=A
  Voltage Sensor1 : fl_lib/Electrical/Electrical Sensors/Voltage Sensor
  Voltage Sensor2 : fl_lib/Electrical/Electrical Sensors/Voltage Sensor
  dclink_measure : Subsystem
  driver_board_c : Subsystem
  isc_dbc : nesl_utility/PS-Simulink Converter  PhysicalDomain=network_engine_domain  SubClassName=ps_output  LeftPortType=input  RightPortType=output  PseudoPeriodic=off  Frequencies=[]  VectorFormat=1-D array  Unit=A  AffineConversion=off
  modulator : Subsystem
  solid_state_inverter : Subsystem
  ugc_dbc : nesl_utility/PS-Simulink Converter  PhysicalDomain=network_engine_domain  SubClassName=ps_output  LeftPortType=input  RightPortType=output  PseudoPeriodic=off  Frequencies=[]  VectorFormat=1-D array  Unit=V  AffineConversion=off
  us_c : PMIOPort  Side=Left
  Udc(+) : PMIOPort  Port=2  Side=Right
  Udc(-) : PMIOPort  Port=3  Side=Right
  tag scope: isc_dbc=global, ugc_dbc=global
  wires:
  driver_board_c/1(us_alphabeta_ctrl) -> modulator/1(u_alphabeta_ctrl)
  ugc_dbc/1 -> [ugc_dbc]  "ugc_dbc"
  isc_dbc/1 -> [isc_dbc]  "isc_dbc"
  connections:
  Voltage Sensor2/RConn1 -- dclink_measure/LConn1
  Capacitor/LConn1 -- Udc(+)/RConn1 -- Voltage Sensor2/LConn1 -- solid_state_inverter/LConn1
  Capacitor/RConn1 -- Udc(-)/RConn1 -- Voltage Sensor2/RConn2 -- solid_state_inverter/LConn2
  Voltage Sensor1/LConn1 -- LFu3/RConn1 -- us_c/RConn1
  Voltage Sensor1/RConn1 -- ugc_dbc/LConn1
  Electrical Reference/LConn1 -- Voltage Sensor1/RConn2
  Current Sensor1/LConn1 -- solid_state_inverter/RConn1
  isc_dbc/LConn1 -- Current Sensor1/RConn1
  Current Sensor1/RConn2 -- LFu3/LConn1

== system afe_rst_inv_psm_distributed_control_two_delays/FRT-VDE4110/FRT-Detection ==
  Abs : Abs  SaturateOnIntegerOverflow=off
  Abs1 : Abs  SaturateOnIntegerOverflow=off
  Constant : Constant  Value=0
  Constant1 : Constant  Value=0
  LVRT_detector : MATLAB Function  TreatAsAtomicUnit=on  SystemSampleTime=ts_afe
  Step3 : Step  Time=settle_time  SampleTime=ts_afe
  dvxi_n/dt : Subsystem
  dvxi_p/dt : Subsystem
  frt_exceeded : Outport
  frt_state : Outport  Port=2
  frt_active : Outport  Port=3
  pwr_lim_enable : Outport  Port=4
  wires:
  [v_grid_neg_xi_avg] -> dvxi_n/dt/1(x), LVRT_detector/2(vxi_n)  "vxi_n"
  [v_grid_pos_xi_avg] -> LVRT_detector/1(vxi_p), dvxi_p/dt/1(x)  "vxi_p"
  [v_grid_neg_eta_avg] -> LVRT_detector/3(veta_n)  "veta_n"
  Step3/1 -> LVRT_detector/6(enable)
  dvxi_p/dt/1(xdot_hat) -> Abs/1
  LVRT_detector/1(pwr_lim_enable) -> pwr_lim_enable/1  "pwr_lim_enable"
  dvxi_n/dt/1(xdot_hat) -> Abs1/1
  Constant/1 -> LVRT_detector/8(reset)
  Constant1/1 -> LVRT_detector/7(red_dyn_enabled)
  LVRT_detector/2(frt_exceeded) -> frt_exceeded/1  "lvrt_exceeded"
  LVRT_detector/4(frt_state) -> frt_state/1
  LVRT_detector/3(frt_active) -> frt_active/1
  Abs/1 -> LVRT_detector/4(vxi_p_dot)  "vxi_p_dot"
  Abs1/1 -> LVRT_detector/5(vxi_n_dot)  "vxi_n_dor"

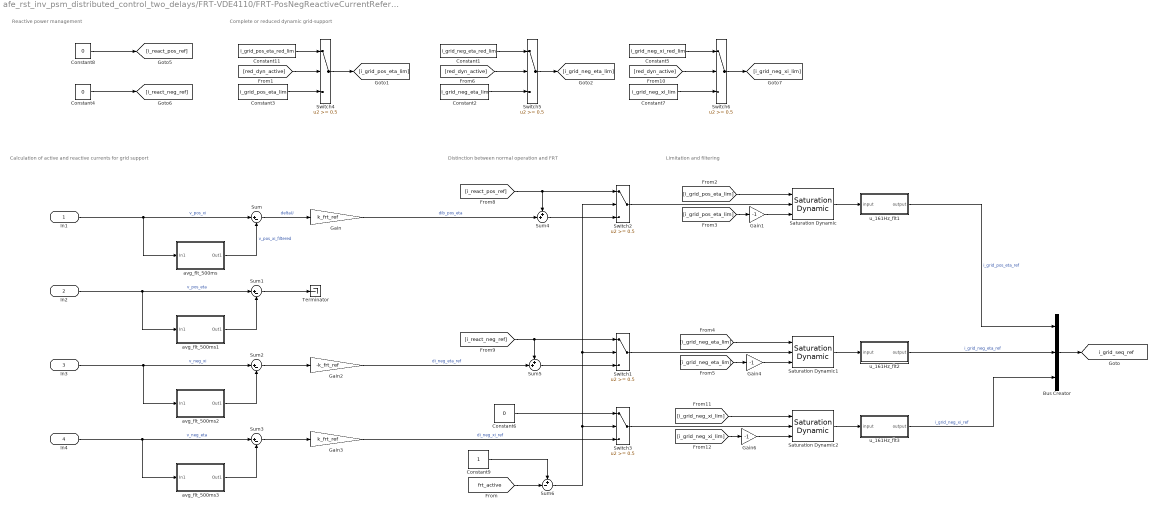
== system afe_rst_inv_psm_distributed_control_two_delays/FRT-VDE4110/FRT-PosNegReactiveCurrentReferences ==
  note: Reactive power management
  note: Distinction between normal operation and FRT
  note: Calculation of active and reactive currents for grid support
  note: Complete or reduced dynamic grid-support
  note: Limitation and filtering
  In1 : Inport
  In2 : Inport  Port=2
  In3 : Inport  Port=3
  In4 : Inport  Port=4
  Bus Creator : BusCreator  Inputs=3
  Constant1 : Constant  Value=i_grid_neg_eta_red_lim
  Constant11 : Constant  Value=i_grid_pos_eta_red_lim
  Constant2 : Constant  Value=i_grid_neg_eta_lim
  Constant3 : Constant  Value=i_grid_pos_eta_lim
  Constant4 : Constant  Value=0
  Constant5 : Constant  Value=i_grid_neg_xi_red_lim
  Constant6 : Constant  Value=0
  Constant7 : Constant  Value=i_grid_neg_xi_lim
  Constant8 : Constant  Value=0
  Constant9 : Constant
  Gain : Gain  Gain=k_frt_ref
  Gain1 : Gain  Gain=-1
  Gain2 : Gain  Gain=-k_frt_ref
  Gain3 : Gain  Gain=k_frt_ref
  Gain4 : Gain  Gain=-1
  Gain6 : Gain  Gain=-1
  Saturation Dynamic : sl_discontinuities/Saturation Dynamic  OutMin=[]  OutMax=[]  OutDataTypeStr=Inherit: Same as second input  OutDataType=fixdt(1, 16)  OutScaling=2^-10  DoSatur=off
  Saturation Dynamic1 : sl_discontinuities/Saturation Dynamic  OutMin=[]  OutMax=[]  OutDataTypeStr=Inherit: Same as second input  OutDataType=fixdt(1, 16)  OutScaling=2^-10  DoSatur=off
  Saturation Dynamic2 : sl_discontinuities/Saturation Dynamic  OutMin=[]  OutMax=[]  OutDataTypeStr=Inherit: Same as second input  OutDataType=fixdt(1, 16)  OutScaling=2^-10  DoSatur=off
  Sum{,1..3} (4 alike) : Sum  Inputs=|+-
  Sum4 : Sum  Inputs=++|
  Sum5 : Sum  Inputs=++|
  Sum6 : Sum  Inputs=+-|
  Switch{1..6} (6 alike) : Switch  Threshold=0.5  SaturateOnIntegerOverflow=off  InputSameDT=off
  Terminator : Terminator
  avg_flt_500ms : Subsystem
  avg_flt_500ms1 : Subsystem
  avg_flt_500ms2 : Subsystem
  avg_flt_500ms3 : Subsystem
  u_161Hz_flt1 : Subsystem
  u_161Hz_flt2 : Subsystem
  u_161Hz_flt3 : Subsystem
  tag scope: i_grid_seq_ref=global
  wires:
  In1/1 -> avg_flt_500ms/1(In1), Sum/1  "v_pos_xi"
  avg_flt_500ms/1(Out1) -> Sum/2  "v_pos_xi_filtered"
  Sum/1 -> Gain/1  "deltaU"
  Sum1/1 -> Terminator/1
  avg_flt_500ms1/1(Out1) -> Sum1/2
  In2/1 -> avg_flt_500ms1/1(In1), Sum1/1  "v_pos_eta"
  avg_flt_500ms3/1(Out1) -> Sum3/2
  Sum2/1 -> Gain2/1
  In3/1 -> avg_flt_500ms2/1(In1), Sum2/1  "v_neg_xi"
  avg_flt_500ms2/1(Out1) -> Sum2/2
  In4/1 -> avg_flt_500ms3/1(In1), Sum3/1  "v_neg_eta"
  Bus Creator/1 -> [i_grid_seq_ref]
  Gain/1 -> Sum4/2  "dib_pos_eta"
  [i_react_pos_ref] -> Switch2/1, Sum4/1
  Sum4/1 -> Switch2/3
  Switch2/1 -> Saturation Dynamic/2
  Saturation Dynamic/1 -> u_161Hz_flt1/1(input)
  Constant6/1 -> Switch3/1
  Gain3/1 -> Switch3/3  "di_neg_xi_ref"
  Sum6/1 -> Switch1/2, Switch2/2, Switch3/2
  Sum3/1 -> Gain3/1
  Gain2/1 -> Sum5/2  "di_neg_eta_ref"
  Sum5/1 -> Switch1/3
  [i_react_neg_ref] -> Switch1/1, Sum5/1
  Switch4/1 -> [i_grid_pos_eta_lim]
  [red_dyn_active] -> Switch4/2
  Constant3/1 -> Switch4/3
  Constant11/1 -> Switch4/1
  [i_grid_pos_eta_lim] -> Saturation Dynamic/1
  [i_grid_pos_eta_lim] -> Gain1/1
  Gain1/1 -> Saturation Dynamic/3
  Saturation Dynamic2/1 -> u_161Hz_flt3/1(input)
  Switch3/1 -> Saturation Dynamic2/2
  [i_grid_neg_xi_lim] -> Saturation Dynamic2/1
  [i_grid_neg_xi_lim] -> Gain6/1
  Gain4/1 -> Saturation Dynamic1/3
  [i_grid_neg_eta_lim] -> Gain4/1
  [i_grid_neg_eta_lim] -> Saturation Dynamic1/1
  Switch1/1 -> Saturation Dynamic1/2
  Saturation Dynamic1/1 -> u_161Hz_flt2/1(input)
  [red_dyn_active] -> Switch5/2
  Constant2/1 -> Switch5/3
  Constant1/1 -> Switch5/1
  Switch5/1 -> [i_grid_neg_eta_lim]
  Constant4/1 -> [i_react_neg_ref]
  Constant8/1 -> [i_react_pos_ref]
  Constant7/1 -> Switch6/3
  Switch6/1 -> [i_grid_neg_xi_lim]
  Constant5/1 -> Switch6/1
  [red_dyn_active] -> Switch6/2
  Gain6/1 -> Saturation Dynamic2/3
  u_161Hz_flt2/1(output) -> Bus Creator/2  "i_grid_neg_eta_ref"
  u_161Hz_flt3/1(output) -> Bus Creator/3  "i_grid_neg_xi_ref"
  u_161Hz_flt1/1(output) -> Bus Creator/1  "i_grid_pos_eta_ref"
  [frt_active] -> Sum6/2
  Constant9/1 -> Sum6/1

== system afe_rst_inv_psm_distributed_control_two_delays/INV-Modular/inv_leg_u ==
  Current Sensor1 : fl_lib/Electrical/Electrical Sensors/Current Sensor
  Electrical Reference : fl_lib/Electrical/Electrical Elements/Electrical Reference
  LFi_1 : fl_lib/Electrical/Electrical Elements/Inductor  l=LFi H  r=RLFi Ohm  g=1e-9 1/Ohm  i_specify=on  i_priority=High  i=0 A  i_nominal_specify=off  i_nominal_value=1  i_nominal_unit=A  v_specify=off  v_priority=None  v=0 V  v_nominal_specify=off  v_nominal_value=1  v_nominal_unit=V  i_L_specify=off  i_L_priority=High  i_L=0 A  i_L_nominal_specify=off  i_L_nominal_value=1  i_L_nominal_unit=A
  Voltage Sensor1 : fl_lib/Electrical/Electrical Sensors/Voltage Sensor
  Voltage Sensor2 : fl_lib/Electrical/Electrical Sensors/Voltage Sensor
  dclink_measure : Subsystem
  driver_board_u : Subsystem
  isu_inv : nesl_utility/PS-Simulink Converter  PhysicalDomain=network_engine_domain  SubClassName=ps_output  LeftPortType=input  RightPortType=output  PseudoPeriodic=off  Frequencies=[]  VectorFormat=1-D array  Unit=A  AffineConversion=off
  modulator : Subsystem
  solid_state_inverter : Subsystem
  us_phase_u_inv : nesl_utility/PS-Simulink Converter  PhysicalDomain=network_engine_domain  SubClassName=ps_output  LeftPortType=input  RightPortType=output  PseudoPeriodic=off  Frequencies=[]  VectorFormat=1-D array  Unit=V  AffineConversion=off
  us_u : PMIOPort  Side=Left
  Udc(+) : PMIOPort  Port=2  Side=Right
  Udc(-) : PMIOPort  Port=3  Side=Right
  tag scope: isu_dbu=global, usu_dbu=global
  wires:
  us_phase_u_inv/1 -> [usu_dbu]  "us_phase_u_inv"
  isu_inv/1 -> [isu_dbu]  "isu_inv"
  driver_board_u/1(us_alphabeta_ctrl) -> modulator/1(us_alphabeta_ctrl)
  connections:
  Voltage Sensor1/RConn1 -- us_phase_u_inv/LConn1
  Electrical Reference/LConn1 -- Voltage Sensor1/RConn2
  isu_inv/LConn1 -- Current Sensor1/RConn1
  Current Sensor1/RConn2 -- LFi_1/RConn1
  Current Sensor1/LConn1 -- Voltage Sensor1/LConn1 -- solid_state_inverter/RConn1
  LFi_1/LConn1 -- us_u/RConn1
  Udc(-)/RConn1 -- Voltage Sensor2/RConn2 -- solid_state_inverter/LConn2
  Udc(+)/RConn1 -- solid_state_inverter/LConn1 -- Voltage Sensor2/LConn1
  Voltage Sensor2/RConn1 -- dclink_measure/LConn1

== system afe_rst_inv_psm_distributed_control_two_delays/INV-Modular/inv_leg_v ==
  Current Sensor1 : fl_lib/Electrical/Electrical Sensors/Current Sensor
  Electrical Reference : fl_lib/Electrical/Electrical Elements/Electrical Reference
  LFi_2 : fl_lib/Electrical/Electrical Elements/Inductor  l=LFi H  r=RLFi Ohm  g=1e-9 1/Ohm  i_specify=on  i_priority=High  i=0 A  i_nominal_specify=off  i_nominal_value=1  i_nominal_unit=A  v_specify=off  v_priority=None  v=0 V  v_nominal_specify=off  v_nominal_value=1  v_nominal_unit=V  i_L_specify=off  i_L_priority=High  i_L=0 A  i_L_nominal_specify=off  i_L_nominal_value=1  i_L_nominal_unit=A
  Voltage Sensor1 : fl_lib/Electrical/Electrical Sensors/Voltage Sensor
  Voltage Sensor2 : fl_lib/Electrical/Electrical Sensors/Voltage Sensor
  dclink_measure : Subsystem
  driver_board_v : Subsystem
  isv_inv : nesl_utility/PS-Simulink Converter  PhysicalDomain=network_engine_domain  SubClassName=ps_output  LeftPortType=input  RightPortType=output  PseudoPeriodic=off  Frequencies=[]  VectorFormat=1-D array  Unit=A  AffineConversion=off
  modulator : Subsystem
  solid_state_inverter : Subsystem
  us_phase_v_inv : nesl_utility/PS-Simulink Converter  PhysicalDomain=network_engine_domain  SubClassName=ps_output  LeftPortType=input  RightPortType=output  PseudoPeriodic=off  Frequencies=[]  VectorFormat=1-D array  Unit=V  AffineConversion=off
  us_v : PMIOPort  Side=Left
  Udc(+) : PMIOPort  Port=2  Side=Right
  Udc(-) : PMIOPort  Port=3  Side=Right
  tag scope: isv_dbv=global, usv_dbv=global
  wires:
  driver_board_v/1(us_alphabeta_ctrl) -> modulator/1(us_alphabeta_ctrl)
  isv_inv/1 -> [isv_dbv]  "isv_inv"
  us_phase_v_inv/1 -> [usv_dbv]  "us_phase_v_inv"
  connections:
  Udc(+)/RConn1 -- Voltage Sensor2/LConn1 -- solid_state_inverter/LConn1
  Udc(-)/RConn1 -- Voltage Sensor2/RConn2 -- solid_state_inverter/LConn2
  LFi_2/LConn1 -- us_v/RConn1
  solid_state_inverter/RConn1 -- Voltage Sensor1/LConn1 -- Current Sensor1/LConn1
  Current Sensor1/RConn2 -- LFi_2/RConn1
  isv_inv/LConn1 -- Current Sensor1/RConn1
  Electrical Reference/LConn1 -- Voltage Sensor1/RConn2
  Voltage Sensor1/RConn1 -- us_phase_v_inv/LConn1
  Voltage Sensor2/RConn1 -- dclink_measure/LConn1

== system afe_rst_inv_psm_distributed_control_two_delays/INV-Modular/inv_leg_w ==
  Current Sensor1 : fl_lib/Electrical/Electrical Sensors/Current Sensor
  Electrical Reference : fl_lib/Electrical/Electrical Elements/Electrical Reference
  LFu3 : fl_lib/Electrical/Electrical Elements/Inductor  l=LFi H  r=RLFi Ohm  g=1e-9 1/Ohm  i_specify=on  i_priority=High  i=0 A  i_nominal_specify=off  i_nominal_value=1  i_nominal_unit=A  v_specify=off  v_priority=None  v=0 V  v_nominal_specify=off  v_nominal_value=1  v_nominal_unit=V  i_L_specify=off  i_L_priority=High  i_L=0 A  i_L_nominal_specify=off  i_L_nominal_value=1  i_L_nominal_unit=A
  Voltage Sensor1 : fl_lib/Electrical/Electrical Sensors/Voltage Sensor
  Voltage Sensor2 : fl_lib/Electrical/Electrical Sensors/Voltage Sensor
  dclink_measure : Subsystem
  driver_board_w : Subsystem
  isw_dbw : nesl_utility/PS-Simulink Converter  PhysicalDomain=network_engine_domain  SubClassName=ps_output  LeftPortType=input  RightPortType=output  PseudoPeriodic=off  Frequencies=[]  VectorFormat=1-D array  Unit=A  AffineConversion=off
  modulator : Subsystem
  solid_state_inverter : Subsystem
  usw_dbw : nesl_utility/PS-Simulink Converter  PhysicalDomain=network_engine_domain  SubClassName=ps_output  LeftPortType=input  RightPortType=output  PseudoPeriodic=off  Frequencies=[]  VectorFormat=1-D array  Unit=V  AffineConversion=off
  us_w : PMIOPort  Side=Left
  Udc(+) : PMIOPort  Port=2  Side=Right
  Udc(-) : PMIOPort  Port=3  Side=Right
  tag scope: isw_dbw=global, usw_dbw=global
  wires:
  isw_dbw/1 -> [isw_dbw]  "isw_dbw"
  usw_dbw/1 -> [usw_dbw]  "usw_dbw"
  driver_board_w/1(us_alphabeta_ctrl) -> modulator/1(u_alphabeta_ctrl)
  connections:
  Current Sensor1/RConn2 -- LFu3/LConn1
  isw_dbw/LConn1 -- Current Sensor1/RConn1
  Current Sensor1/LConn1 -- solid_state_inverter/RConn1
  Electrical Reference/LConn1 -- Voltage Sensor1/RConn2
  Voltage Sensor1/RConn1 -- usw_dbw/LConn1
  us_w/RConn1 -- LFu3/RConn1 -- Voltage Sensor1/LConn1
  Udc(-)/RConn1 -- Voltage Sensor2/RConn2 -- solid_state_inverter/LConn2
  Udc(+)/RConn1 -- Voltage Sensor2/LConn1 -- solid_state_inverter/LConn1
  Voltage Sensor2/RConn1 -- dclink_measure/LConn1
